simulink model "SAPF_pq0_theory"  (R2025a)
settings: Solver=VariableStepAuto  StartTime=0.0  StopTime=0.5  RelTol=1e-3
libraries: fl_lib x16, nesl_utility x16, ee_lib x12, mcbeeMathTransformLib x2, eeGeneralControl x1
settings Model: Creator=nahiz  LastModifiedBy=18023021
settings SimscapeCC: SimscapeNominalValues="[{\"value\":\"1\",\"unit\":\"A\"},{\"value\":\"1\",\"unit\":\"bar\"},{\"value\":\"1\",\"unit\":\"cm^2\"},{\"value\":\"1\",\"unit\":\"cm^3/s\"},{\"value\":\"1\",\"unit\":\"kJ/kg\"},{\"value\":\"1\",\"unit\":\"kW\"},{\"value\":\"1\",\"unit\":\"l\"},{\"value\":\"1\",\"unit\":\"N\"},{\"value\":\"1\",\"unit\":\"N*m\"},{\"value\":\"1\",\"unit\":\"V\"},{\"value\":\"0.001\",\"unit\":\"Wb\"}]"  SimscapeLogType=all  SimscapeLogDataHistory=10000.0

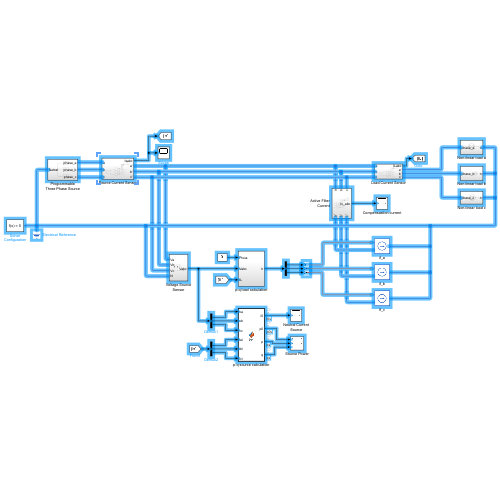
[thumbnail: Simulink's stored preview of the top-level diagram]
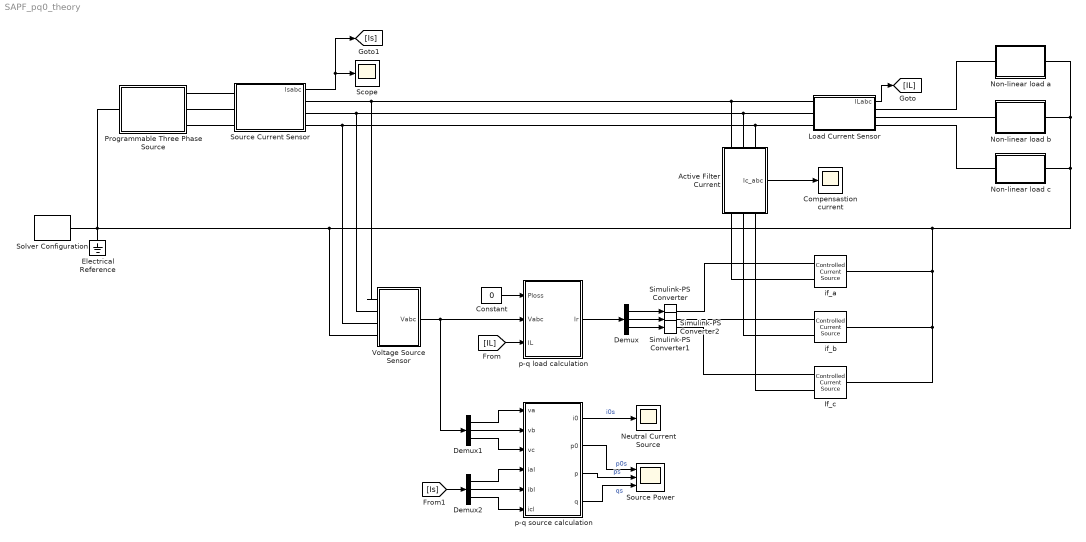
== system SAPF_pq0_theory ==
  Active Filter Current : Subsystem
      settings: PortSchema="{\"entries\":[{\"content\":{\"sides\":[{\"content\":{\"connectorIds\":[\"LConn1\",\"LConn2\",\"LConn3\"]},\"type\":\"ConnectorPlacement.EquallySpacedRectSide\",\"uuid\":\"e0b89ca1-2dce-4101-8bbe-782629a672ac\"},{\"content\":{\"connectorIds\":[\"RConn1\",\"RConn2\",\"RConn3\"],\"side\":\"RIGHT\"},\"type\":\"ConnectorPlacement.EquallySpacedRectSide\",\"uuid\":\"01d628be-6f4d-45a1-9eca-35615a86d2be\"},{\"content\":{\"side\":\"TOP\"},\"type\":\"ConnectorPlacement.EquallySpacedRectSide\",\"uuid\":\"f08109ad-0e21-41b9-b238-385b9ba1e634\"},{\"content\":{\"connectorIds\":[\"Out1\"],\"side\":\"BOTTOM\"},\"type\":\"ConnectorPlacement.EquallySpacedRectSide\",\"uuid\":\"6980f4f4-e67c-41c5-899b-6138d1e73cf4\"}]},\"type\":\"ConnectorPlacement.EquallySpacedConnector\",\"uuid\":\"23e52943-ee20-486d-b1d7-7933c9cd5a10\"}],\"packageUris\":[\"http://schema.mathworks.com/mf0/Connector/R2020b\"],\"version\":\"1.0\"}"
  Compensastion current : Scope
      settings: DataLoggingVariableName=ScopeData3
  Constant : Constant  Value=0
  Demux : Demux  Outputs=3
  Demux1 : Demux  Outputs=3
  Demux2 : Demux  Outputs=3
  Electrical Reference : fl_lib/Electrical/Electrical Elements/Electrical Reference
  If_c : fl_lib/Electrical/Electrical Sources/Controlled Current Source
  Load Current Sensor : Subsystem
  Neutral Current Source : Scope
      settings: DataLoggingVariableName=ScopeData4
  Non-linear load a : Subsystem
  Non-linear load b : Subsystem
  Non-linear load c : Subsystem
  Programmable Three Phase Source : Subsystem
  Scope : Scope
  Simulink-PS Converter : nesl_utility/Simulink-PS Converter  PhysicalDomain=network_engine_domain  SubClassName=ps_input  LeftPortType=input  RightPortType=output  PseudoPeriodic=off  Frequencies=[]  NoiseDistribution=none  NoiseParameters=[]  Unit=1  AffineConversion=off  FilteringAndDerivatives=zero  SimscapeFilterOrder=1  InputFilterTimeConstant=0.001  UdotUserProvided=0
  Simulink-PS Converter1 : nesl_utility/Simulink-PS Converter  PhysicalDomain=network_engine_domain  SubClassName=ps_input  LeftPortType=input  RightPortType=output  PseudoPeriodic=off  Frequencies=[]  NoiseDistribution=none  NoiseParameters=[]  Unit=1  AffineConversion=off  FilteringAndDerivatives=zero  SimscapeFilterOrder=1  InputFilterTimeConstant=0.001  UdotUserProvided=0
  Simulink-PS Converter2 : nesl_utility/Simulink-PS Converter  PhysicalDomain=network_engine_domain  SubClassName=ps_input  LeftPortType=input  RightPortType=output  PseudoPeriodic=off  Frequencies=[]  NoiseDistribution=none  NoiseParameters=[]  Unit=1  AffineConversion=off  FilteringAndDerivatives=zero  SimscapeFilterOrder=1  InputFilterTimeConstant=0.001  UdotUserProvided=0
  Solver Configuration : nesl_utility/Solver Configuration  PhysicalDomain=network_engine_domain  SubClassName=solver  LeftPortType=input  RightPortType=generic  Tones=[]  Harmonics=[]  SimulateNoise=off  Profile=off  UseLocalSampling=off  EnableSwitchedLinearOptims=on  FrequencyDomain=off  UseCCode=off  RelTol=0.001  AbsTol=0.001  MinStep=1e-09  ToWorkspace=off  RevertToSquareIcSolve=off  NumHomotopyIterations=100  PhasorMode=off  PhasorModeNumHarmonics=1  ConsistencySolver=NEWTON_XTOL_AFTER_FTOL  IndexReductionMethod=DerivativeReplacement  DoDC=off  ResidualTolerance=1e-09  ConsistencyTolSource=GLOBAL  ConsistencyAbsTol=0.001  ConsistencyRelTol=0.001  ConsistencyTolFactor=0.001  UseLocalSolver=off  LocalSolverChoice=NE_BACKWARD_EULER_ADVANCER  ResolveIndetEquations=on  FunctionEvalNumThread=1  LocalSolverSampleTime=0.001  DoFixedCost=off  MaxNonlinIter=3  MaxModeIter=2  ComputeImpulses=off  ImpulseIterations=2  LinearAlgebra=auto  LinearAlgebraNumThread=0  EquationFormulation=NE_TIME_EF  DelaysMemoryBudget=1024  AutomaticFiltering=on  FilteringTimeConstant=0.001  PartitionStorageMethod=AS_NEEDED  PartitionMemoryBudget=1024  PartitionMethod=ROBUST  MultibodyUseLocalSolver=off  MultibodyLocalSolverChoice=ODE1  MultibodyLocalSolverSampleTime=0.001
  Source Current Sensor : Subsystem
  Source Power : Scope  NumInputPorts=3
      settings: ActiveDisplayYMinimum=-299.915797041433  ActiveDisplayYMaximum=2699.2421733727761  DataLoggingVariableName=ScopeData2
  Voltage Source Sensor : Subsystem
  if_a : fl_lib/Electrical/Electrical Sources/Controlled Current Source
  if_b : fl_lib/Electrical/Electrical Sources/Controlled Current Source
  p-q load calculation : Subsystem
  p-q source calculation : MATLAB Function  TreatAsAtomicUnit=on
  wires:
  Load Current Sensor/1(ILabc) -> [IL]
  Source Current Sensor/1(Isabc) -> [Is], Scope/1
  Voltage Source Sensor/1(Vabc) -> Demux1/1, p-q load calculation/2(Vabc)
  p-q load calculation/1(Ir) -> Demux/1
  Constant/1 -> p-q load calculation/1(Ploss)
  [IL] -> p-q load calculation/3(IL)
  Demux/1 -> Simulink-PS Converter/1
  Demux/2 -> Simulink-PS Converter1/1
  Demux/3 -> Simulink-PS Converter2/1
  Demux1/1 -> p-q source calculation/1(va)
  Demux1/2 -> p-q source calculation/2(vb)
  Demux1/3 -> p-q source calculation/3(vc)
  [Is] -> Demux2/1
  Demux2/1 -> p-q source calculation/4(ial)
  Demux2/2 -> p-q source calculation/5(ibl)
  Demux2/3 -> p-q source calculation/6(icl)
  p-q source calculation/1(i0) -> Neutral Current Source/1  "i0s"
  p-q source calculation/2(p0) -> Source Power/1  "p0s"
  p-q source calculation/3(p) -> Source Power/2  "ps"
  p-q source calculation/4(q) -> Source Power/3  "qs"
  Active Filter Current/1(Ic_abc) -> Compensastion current/1
  connections:
  Active Filter Current/LConn3 -- Voltage Source Sensor/LConn3 -- Source Current Sensor/RConn3 -- Load Current Sensor/LConn3
  Active Filter Current/LConn2 -- Voltage Source Sensor/LConn2 -- Source Current Sensor/RConn2 -- Load Current Sensor/LConn2
  Programmable Three Phase Source/RConn1 -- Solver Configuration/RConn1 -- Electrical Reference/LConn1 -- Voltage Source Sensor/LConn4 -- Non-linear load b/RConn1 -- Non-linear load a/RConn1 -- Non-linear load c/RConn1 -- If_c/LConn1 -- if_b/LConn1 -- if_a/LConn1
  Active Filter Current/LConn1 -- Voltage Source Sensor/LConn1 -- Source Current Sensor/RConn1 -- Load Current Sensor/LConn1
  if_b/RConn2 -- Active Filter Current/RConn2
  if_a/RConn2 -- Active Filter Current/RConn1
  Programmable Three Phase Source/LConn2 -- Source Current Sensor/LConn2
  Programmable Three Phase Source/LConn1 -- Source Current Sensor/LConn1
  Programmable Three Phase Source/LConn3 -- Source Current Sensor/LConn3
  If_c/RConn2 -- Active Filter Current/RConn3
  Simulink-PS Converter/RConn1 -- if_a/RConn1
  Simulink-PS Converter1/RConn1 -- if_b/RConn1
  Simulink-PS Converter2/RConn1 -- If_c/RConn1
  Load Current Sensor/RConn3 -- Non-linear load c/LConn1
  Load Current Sensor/RConn2 -- Non-linear load b/LConn1
  Load Current Sensor/RConn1 -- Non-linear load a/LConn1

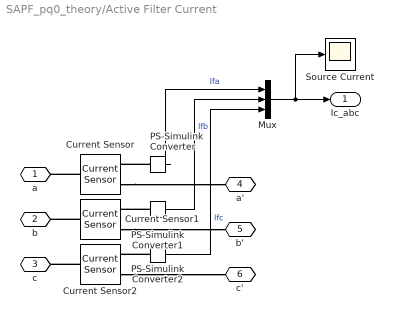
== system SAPF_pq0_theory/Active Filter Current ==
  Current Sensor : fl_lib/Electrical/Electrical Sensors/Current Sensor
  Current Sensor1 : fl_lib/Electrical/Electrical Sensors/Current Sensor
  Current Sensor2 : fl_lib/Electrical/Electrical Sensors/Current Sensor
  Mux : Mux  Inputs=3
  PS-Simulink Converter : nesl_utility/PS-Simulink Converter  PhysicalDomain=network_engine_domain  SubClassName=ps_output  LeftPortType=input  RightPortType=output  PseudoPeriodic=off  Frequencies=[]  VectorFormat=inherit  Unit=inherit  AffineConversion=off
  PS-Simulink Converter1 : nesl_utility/PS-Simulink Converter  PhysicalDomain=network_engine_domain  SubClassName=ps_output  LeftPortType=input  RightPortType=output  PseudoPeriodic=off  Frequencies=[]  VectorFormat=inherit  Unit=inherit  AffineConversion=off
  PS-Simulink Converter2 : nesl_utility/PS-Simulink Converter  PhysicalDomain=network_engine_domain  SubClassName=ps_output  LeftPortType=input  RightPortType=output  PseudoPeriodic=off  Frequencies=[]  VectorFormat=inherit  Unit=inherit  AffineConversion=off
  Source Current : Scope
  a : PMIOPort  Side=Left
  b : PMIOPort  Port=2  Side=Left
  c : PMIOPort  Port=3  Side=Left
  a' : PMIOPort  Port=4  Side=Right
  b' : PMIOPort  Port=5  Side=Right
  c' : PMIOPort  Port=6  Side=Right
  Ic_abc : Outport
  wires:
  PS-Simulink Converter1/1 -> Mux/2  "Ifb"
  PS-Simulink Converter/1 -> Mux/1  "Ifa"
  PS-Simulink Converter2/1 -> Mux/3  "Ifc"
  Mux/1 -> Source Current/1, Ic_abc/1
  connections:
  PS-Simulink Converter2/LConn1 -- Current Sensor2/RConn1
  PS-Simulink Converter1/LConn1 -- Current Sensor1/RConn1
  Current Sensor/LConn1 -- a/RConn1
  PS-Simulink Converter/LConn1 -- Current Sensor/RConn1
  Current Sensor2/LConn1 -- c/RConn1
  Current Sensor1/LConn1 -- b/RConn1
  Current Sensor/RConn2 -- a'/RConn1
  Current Sensor1/RConn2 -- b'/RConn1
  Current Sensor2/RConn2 -- c'/RConn1

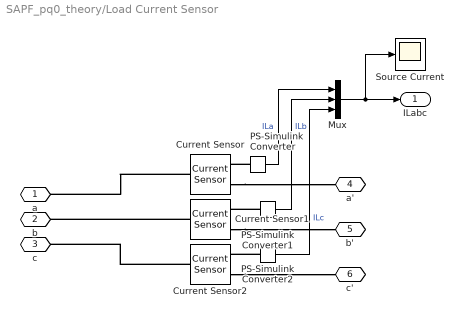
== system SAPF_pq0_theory/Load Current Sensor ==
  Current Sensor : fl_lib/Electrical/Electrical Sensors/Current Sensor
  Current Sensor1 : fl_lib/Electrical/Electrical Sensors/Current Sensor
  Current Sensor2 : fl_lib/Electrical/Electrical Sensors/Current Sensor
  Mux : Mux  Inputs=3
  PS-Simulink Converter : nesl_utility/PS-Simulink Converter  PhysicalDomain=network_engine_domain  SubClassName=ps_output  LeftPortType=input  RightPortType=output  PseudoPeriodic=off  Frequencies=[]  VectorFormat=inherit  Unit=inherit  AffineConversion=off
  PS-Simulink Converter1 : nesl_utility/PS-Simulink Converter  PhysicalDomain=network_engine_domain  SubClassName=ps_output  LeftPortType=input  RightPortType=output  PseudoPeriodic=off  Frequencies=[]  VectorFormat=inherit  Unit=inherit  AffineConversion=off
  PS-Simulink Converter2 : nesl_utility/PS-Simulink Converter  PhysicalDomain=network_engine_domain  SubClassName=ps_output  LeftPortType=input  RightPortType=output  PseudoPeriodic=off  Frequencies=[]  VectorFormat=inherit  Unit=inherit  AffineConversion=off
  Source Current : Scope
  a : PMIOPort  Side=Left
  b : PMIOPort  Port=2  Side=Left
  c : PMIOPort  Port=3  Side=Left
  a' : PMIOPort  Port=4  Side=Right
  b' : PMIOPort  Port=5  Side=Right
  c' : PMIOPort  Port=6  Side=Right
  ILabc : Outport
  wires:
  PS-Simulink Converter1/1 -> Mux/2  "ILb"
  PS-Simulink Converter/1 -> Mux/1  "ILa"
  PS-Simulink Converter2/1 -> Mux/3  "ILc"
  Mux/1 -> Source Current/1, ILabc/1
  connections:
  PS-Simulink Converter2/LConn1 -- Current Sensor2/RConn1
  PS-Simulink Converter1/LConn1 -- Current Sensor1/RConn1
  Current Sensor/LConn1 -- a/RConn1
  PS-Simulink Converter/LConn1 -- Current Sensor/RConn1
  Current Sensor2/LConn1 -- c/RConn1
  Current Sensor1/LConn1 -- b/RConn1
  Current Sensor/RConn2 -- a'/RConn1
  Current Sensor1/RConn2 -- b'/RConn1
  Current Sensor2/RConn2 -- c'/RConn1

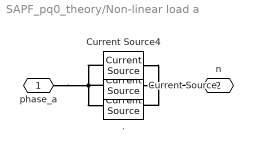
== system SAPF_pq0_theory/Non-linear load a ==
  . : ee_lib/Sources/Current Source  dc_current=0 A  ac_current=1 A  ac_shift=10 deg  ac_frequency=7*50 Hz  noise_mode=ee.enum.sources.noise.Disabled  PSD=0 A^2/Hz  sample_time=1e-3 s  repeatability=ee.enum.sources.repeatability.NotRepeatable  user_seed=0  auto_seed=3516351732  i_specify=off  i_priority=None  i=0 A  i_nominal_specify=off  i_nominal_value=1  i_nominal_unit=A  v_specify=off  v_priority=None  v=0 V  v_nominal_specify=off  v_nominal_value=1  v_nominal_unit=V
  Current Source : ee_lib/Sources/Current Source  dc_current=0 A  ac_current=20 A  ac_shift=10 deg  ac_frequency=50 Hz  noise_mode=ee.enum.sources.noise.Disabled  PSD=0 A^2/Hz  sample_time=1e-3 s  repeatability=ee.enum.sources.repeatability.NotRepeatable  user_seed=0  auto_seed=3127860819  i_specify=off  i_priority=None  i=0 A  i_nominal_specify=off  i_nominal_value=1  i_nominal_unit=A  v_specify=off  v_priority=None  v=0 V  v_nominal_specify=off  v_nominal_value=1  v_nominal_unit=V
  Current Source4 : ee_lib/Sources/Current Source  dc_current=0 A  ac_current=3 A  ac_shift=10 deg  ac_frequency=5*50 Hz  noise_mode=ee.enum.sources.noise.Disabled  PSD=0 A^2/Hz  sample_time=1e-3 s  repeatability=ee.enum.sources.repeatability.NotRepeatable  user_seed=0  auto_seed=810846759  i_specify=off  i_priority=None  i=0 A  i_nominal_specify=off  i_nominal_value=1  i_nominal_unit=A  v_specify=off  v_priority=None  v=0 V  v_nominal_specify=off  v_nominal_value=1  v_nominal_unit=V
  phase_a : PMIOPort  Side=Left
  n : PMIOPort  Port=2  Side=Right
  connections:
  Current Source/LConn1 -- ./LConn1 -- n/RConn1 -- Current Source4/LConn1
  Current Source4/RConn1 -- ./RConn1 -- phase_a/RConn1 -- Current Source/RConn1

== system SAPF_pq0_theory/Non-linear load b ==
  Current Source5 : ee_lib/Sources/Current Source  dc_current=0 A  ac_current=20 A  ac_shift=-130 deg  ac_frequency=50 Hz  noise_mode=ee.enum.sources.noise.Disabled  PSD=0 A^2/Hz  sample_time=1e-3 s  repeatability=ee.enum.sources.repeatability.NotRepeatable  user_seed=0  auto_seed=5147076  i_specify=off  i_priority=None  i=0 A  i_nominal_specify=off  i_nominal_value=1  i_nominal_unit=A  v_specify=off  v_priority=None  v=0 V  v_nominal_specify=off  v_nominal_value=1  v_nominal_unit=V
  Current Source6 : ee_lib/Sources/Current Source  dc_current=0 A  ac_current=1 A  ac_shift=-130 deg  ac_frequency=7*50 Hz  noise_mode=ee.enum.sources.noise.Disabled  PSD=0 A^2/Hz  sample_time=1e-3 s  repeatability=ee.enum.sources.repeatability.NotRepeatable  user_seed=0  auto_seed=1359011463  i_specify=off  i_priority=None  i=0 A  i_nominal_specify=off  i_nominal_value=1  i_nominal_unit=A  v_specify=off  v_priority=None  v=0 V  v_nominal_specify=off  v_nominal_value=1  v_nominal_unit=V
  Current Source7 : ee_lib/Sources/Current Source  dc_current=0 A  ac_current=3 A  ac_shift=-130 deg  ac_frequency=5*50 Hz  noise_mode=ee.enum.sources.noise.Disabled  PSD=0 A^2/Hz  sample_time=1e-3 s  repeatability=ee.enum.sources.repeatability.NotRepeatable  user_seed=0  auto_seed=3004832076  i_specify=off  i_priority=None  i=0 A  i_nominal_specify=off  i_nominal_value=1  i_nominal_unit=A  v_specify=off  v_priority=None  v=0 V  v_nominal_specify=off  v_nominal_value=1  v_nominal_unit=V
  phase_b : PMIOPort  Side=Left
  n : PMIOPort  Port=2  Side=Right
  connections:
  Current Source6/LConn1 -- n/RConn1 -- Current Source7/LConn1 -- Current Source5/LConn1
  Current Source6/RConn1 -- phase_b/RConn1 -- Current Source7/RConn1 -- Current Source5/RConn1

== system SAPF_pq0_theory/Non-linear load c ==
  Current Source1 : ee_lib/Sources/Current Source  dc_current=0 A  ac_current=3 A  ac_shift=110 deg  ac_frequency=5*50 Hz  noise_mode=ee.enum.sources.noise.Disabled  PSD=0 A^2/Hz  sample_time=1e-3 s  repeatability=ee.enum.sources.repeatability.NotRepeatable  user_seed=0  auto_seed=755105624  i_specify=off  i_priority=None  i=0 A  i_nominal_specify=off  i_nominal_value=1  i_nominal_unit=A  v_specify=off  v_priority=None  v=0 V  v_nominal_specify=off  v_nominal_value=1  v_nominal_unit=V
  Current Source2 : ee_lib/Sources/Current Source  dc_current=0 A  ac_current=20 A  ac_shift=110 deg  ac_frequency=50 Hz  noise_mode=ee.enum.sources.noise.Disabled  PSD=0 A^2/Hz  sample_time=1e-3 s  repeatability=ee.enum.sources.repeatability.NotRepeatable  user_seed=0  auto_seed=1547781561  i_specify=off  i_priority=None  i=0 A  i_nominal_specify=off  i_nominal_value=1  i_nominal_unit=A  v_specify=off  v_priority=None  v=0 V  v_nominal_specify=off  v_nominal_value=1  v_nominal_unit=V
  Current Source8 : ee_lib/Sources/Current Source  dc_current=0 A  ac_current=1 A  ac_shift=110 deg  ac_frequency=7*50 Hz  noise_mode=ee.enum.sources.noise.Disabled  PSD=0 A^2/Hz  sample_time=1e-3 s  repeatability=ee.enum.sources.repeatability.NotRepeatable  user_seed=0  auto_seed=2685450550  i_specify=off  i_priority=None  i=0 A  i_nominal_specify=off  i_nominal_value=1  i_nominal_unit=A  v_specify=off  v_priority=None  v=0 V  v_nominal_specify=off  v_nominal_value=1  v_nominal_unit=V
  phase_c : PMIOPort  Side=Left
  n : PMIOPort  Port=2  Side=Right
  connections:
  Current Source8/LConn1 -- Current Source1/LConn1 -- n/RConn1 -- Current Source2/LConn1
  Current Source1/RConn1 -- phase_c/RConn1 -- Current Source8/RConn1 -- Current Source2/RConn1

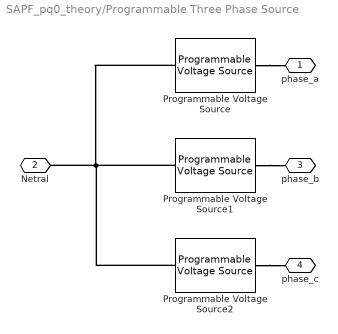
== system SAPF_pq0_theory/Programmable Three Phase Source ==
  Programmable Voltage Source : ee_lib/Sources/Programmable Voltage Source  magnitude_type=ee.enum.timechanging.constant  ac_magnitude=100 V  magn_ramp=1 V/s  magn_step=1 V  magn_modu_magn=1 V  magn_modu_freq=1 Hz  magn_t1=1 s  magn_t2=2 s  frequency_type=ee.enum.timechanging.constant  ac_frequency=50 Hz  freq_ramp=1 Hz/s  freq_step=1 Hz  freq_modu_magn=1 Hz  freq_modu_freq=1 Hz  freq_t1=1 s  freq_t2=2 s  phase_type=ee.enum.timechanging.constant  ac_shift=0 deg  phase_ramp=1 deg/s  phase_step=1 deg  phase_modu_magn=1 deg  phase_modu_freq=1 Hz  phase_t1=1 s  phase_t2=2 s  dc_type=ee.enum.timechanging.constant  dc_voltage=0 V  dc_ramp=1 V/s  dc_step=1 V  dc_modu_magn=1 V  dc_modu_freq=1 Hz  dc_t1=1 s  dc_t2=2 s  harmonic_option=1  harmonic_orders=[5, 7, 11, 13]  harmonic_ratios=[.2, .2, .1, .1]  harmonic_shifts=[0, 0, 0, 0] deg  harmonic_t1=-inf s  harmonic_t2=inf s  noise_mode=0  PSD=0 V^2/Hz  repeatability=1  auto_seed=0  user_seed=0  sample_time=1e-3 s  i_specify=off  i_priority=None  i=0 A  i_nominal_specify=off  i_nominal_value=1  i_nominal_unit=A  v_specify=off  v_priority=None  v=0 V  v_nominal_specify=off  v_nominal_value=1  v_nominal_unit=V
      settings: InternalSimscapePortConfiguration="{\"Bottom\":[],\"Left\":[{\"id\":\"p\",\"label\":\"+\",\"type\":\"foundation.electrical.electrical\"}],\"Right\":[{\"id\":\"n\",\"label\":\"-\",\"type\":\"foundation.electrical.electrical\"}],\"Top\":[]}"
  Programmable Voltage Source1 : ee_lib/Sources/Programmable Voltage Source  magnitude_type=ee.enum.timechanging.constant  ac_magnitude=311 V  magn_ramp=1 V/s  magn_step=1 V  magn_modu_magn=1 V  magn_modu_freq=1 Hz  magn_t1=1 s  magn_t2=2 s  frequency_type=ee.enum.timechanging.constant  ac_frequency=50 Hz  freq_ramp=1 Hz/s  freq_step=1 Hz  freq_modu_magn=1 Hz  freq_modu_freq=1 Hz  freq_t1=1 s  freq_t2=2 s  phase_type=ee.enum.timechanging.constant  ac_shift=-120 deg  phase_ramp=1 deg/s  phase_step=1 deg  phase_modu_magn=1 deg  phase_modu_freq=1 Hz  phase_t1=1 s  phase_t2=2 s  dc_type=ee.enum.timechanging.constant  dc_voltage=0 V  dc_ramp=1 V/s  dc_step=1 V  dc_modu_magn=1 V  dc_modu_freq=1 Hz  dc_t1=1 s  dc_t2=2 s  harmonic_option=1  harmonic_orders=[5, 7, 11, 13]  harmonic_ratios=[.2, .2, .1, .1]  harmonic_shifts=[0, 0, 0, 0] deg  harmonic_t1=-inf s  harmonic_t2=inf s  noise_mode=0  PSD=0 V^2/Hz  repeatability=1  auto_seed=0  user_seed=0  sample_time=1e-3 s  i_specify=off  i_priority=None  i=0 A  i_nominal_specify=off  i_nominal_value=1  i_nominal_unit=A  v_specify=off  v_priority=None  v=0 V  v_nominal_specify=off  v_nominal_value=1  v_nominal_unit=V
      settings: InternalSimscapePortConfiguration="{\"Bottom\":[],\"Left\":[{\"id\":\"p\",\"label\":\"+\",\"type\":\"foundation.electrical.electrical\"}],\"Right\":[{\"id\":\"n\",\"label\":\"-\",\"type\":\"foundation.electrical.electrical\"}],\"Top\":[]}"
  Programmable Voltage Source2 : ee_lib/Sources/Programmable Voltage Source  magnitude_type=ee.enum.timechanging.constant  ac_magnitude=311 V  magn_ramp=1 V/s  magn_step=1 V  magn_modu_magn=1 V  magn_modu_freq=1 Hz  magn_t1=1 s  magn_t2=2 s  frequency_type=ee.enum.timechanging.constant  ac_frequency=50 Hz  freq_ramp=1 Hz/s  freq_step=1 Hz  freq_modu_magn=1 Hz  freq_modu_freq=1 Hz  freq_t1=1 s  freq_t2=2 s  phase_type=ee.enum.timechanging.constant  ac_shift=120 deg  phase_ramp=1 deg/s  phase_step=1 deg  phase_modu_magn=1 deg  phase_modu_freq=1 Hz  phase_t1=1 s  phase_t2=2 s  dc_type=ee.enum.timechanging.constant  dc_voltage=0 V  dc_ramp=1 V/s  dc_step=1 V  dc_modu_magn=1 V  dc_modu_freq=1 Hz  dc_t1=1 s  dc_t2=2 s  harmonic_option=1  harmonic_orders=[5, 7, 11, 13]  harmonic_ratios=[.2, .2, .1, .1]  harmonic_shifts=[0, 0, 0, 0] deg  harmonic_t1=-inf s  harmonic_t2=inf s  noise_mode=0  PSD=0 V^2/Hz  repeatability=1  auto_seed=0  user_seed=0  sample_time=1e-3 s  i_specify=off  i_priority=None  i=0 A  i_nominal_specify=off  i_nominal_value=1  i_nominal_unit=A  v_specify=off  v_priority=None  v=0 V  v_nominal_specify=off  v_nominal_value=1  v_nominal_unit=V
      settings: InternalSimscapePortConfiguration="{\"Bottom\":[],\"Left\":[{\"id\":\"p\",\"label\":\"+\",\"type\":\"foundation.electrical.electrical\"}],\"Right\":[{\"id\":\"n\",\"label\":\"-\",\"type\":\"foundation.electrical.electrical\"}],\"Top\":[]}"
  phase_a : PMIOPort  Side=Left
  Netral : PMIOPort  Port=2  Side=Right
  phase_b : PMIOPort  Port=3  Side=Left
  phase_c : PMIOPort  Port=4  Side=Left
  connections:
  Programmable Voltage Source2/LConn1 -- phase_c/RConn1
  Programmable Voltage Source1/RConn1 -- Programmable Voltage Source2/RConn1 -- Programmable Voltage Source/RConn1 -- Netral/RConn1
  Programmable Voltage Source/LConn1 -- phase_a/RConn1
  Programmable Voltage Source1/LConn1 -- phase_b/RConn1

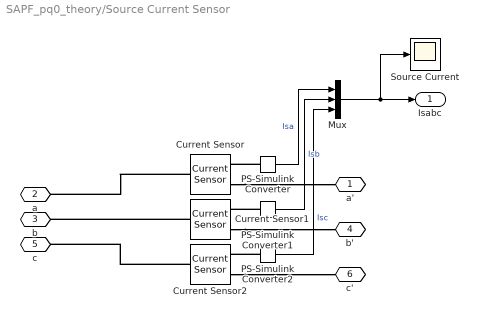
== system SAPF_pq0_theory/Source Current Sensor ==
  Current Sensor : fl_lib/Electrical/Electrical Sensors/Current Sensor
  Current Sensor1 : fl_lib/Electrical/Electrical Sensors/Current Sensor
  Current Sensor2 : fl_lib/Electrical/Electrical Sensors/Current Sensor
  Mux : Mux  Inputs=3
  PS-Simulink Converter : nesl_utility/PS-Simulink Converter  PhysicalDomain=network_engine_domain  SubClassName=ps_output  LeftPortType=input  RightPortType=output  PseudoPeriodic=off  Frequencies=[]  VectorFormat=inherit  Unit=inherit  AffineConversion=off
  PS-Simulink Converter1 : nesl_utility/PS-Simulink Converter  PhysicalDomain=network_engine_domain  SubClassName=ps_output  LeftPortType=input  RightPortType=output  PseudoPeriodic=off  Frequencies=[]  VectorFormat=inherit  Unit=inherit  AffineConversion=off
  PS-Simulink Converter2 : nesl_utility/PS-Simulink Converter  PhysicalDomain=network_engine_domain  SubClassName=ps_output  LeftPortType=input  RightPortType=output  PseudoPeriodic=off  Frequencies=[]  VectorFormat=inherit  Unit=inherit  AffineConversion=off
  Source Current : Scope
  a' : PMIOPort  Side=Right
  a : PMIOPort  Port=2  Side=Left
  b : PMIOPort  Port=3  Side=Left
  b' : PMIOPort  Port=4  Side=Right
  c : PMIOPort  Port=5  Side=Left
  c' : PMIOPort  Port=6  Side=Right
  Isabc : Outport
  wires:
  PS-Simulink Converter1/1 -> Mux/2  "Isb"
  PS-Simulink Converter/1 -> Mux/1  "Isa"
  PS-Simulink Converter2/1 -> Mux/3  "Isc"
  Mux/1 -> Source Current/1, Isabc/1
  connections:
  PS-Simulink Converter2/LConn1 -- Current Sensor2/RConn1
  PS-Simulink Converter1/LConn1 -- Current Sensor1/RConn1
  Current Sensor/LConn1 -- a/RConn1
  PS-Simulink Converter/LConn1 -- Current Sensor/RConn1
  Current Sensor2/LConn1 -- c/RConn1
  Current Sensor1/LConn1 -- b/RConn1
  Current Sensor/RConn2 -- a'/RConn1
  Current Sensor1/RConn2 -- b'/RConn1
  Current Sensor2/RConn2 -- c'/RConn1

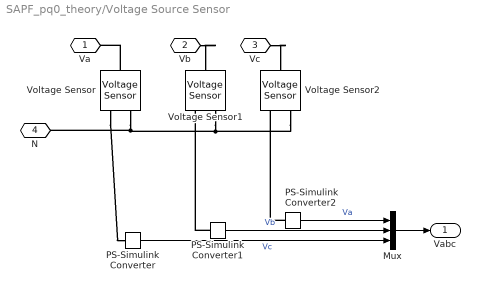
== system SAPF_pq0_theory/Voltage Source Sensor ==
  Mux : Mux  Inputs=3
  PS-Simulink Converter : nesl_utility/PS-Simulink Converter  PhysicalDomain=network_engine_domain  SubClassName=ps_output  LeftPortType=input  RightPortType=output  PseudoPeriodic=off  Frequencies=[]  VectorFormat=inherit  Unit=inherit  AffineConversion=off
  PS-Simulink Converter1 : nesl_utility/PS-Simulink Converter  PhysicalDomain=network_engine_domain  SubClassName=ps_output  LeftPortType=input  RightPortType=output  PseudoPeriodic=off  Frequencies=[]  VectorFormat=inherit  Unit=inherit  AffineConversion=off
  PS-Simulink Converter2 : nesl_utility/PS-Simulink Converter  PhysicalDomain=network_engine_domain  SubClassName=ps_output  LeftPortType=input  RightPortType=output  PseudoPeriodic=off  Frequencies=[]  VectorFormat=inherit  Unit=inherit  AffineConversion=off
  Voltage Sensor : fl_lib/Electrical/Electrical Sensors/Voltage Sensor
  Voltage Sensor1 : fl_lib/Electrical/Electrical Sensors/Voltage Sensor
  Voltage Sensor2 : fl_lib/Electrical/Electrical Sensors/Voltage Sensor
  Va : PMIOPort  Side=Left
  Vb : PMIOPort  Port=2  Side=Left
  Vc : PMIOPort  Port=3  Side=Left
  N : PMIOPort  Port=4  Side=Left
  Vabc : Outport
  wires:
  PS-Simulink Converter/1 -> Mux/3  "Vc"
  PS-Simulink Converter2/1 -> Mux/1  "Va"
  PS-Simulink Converter1/1 -> Mux/2  "Vb"
  Mux/1 -> Vabc/1
  connections:
  PS-Simulink Converter1/LConn1 -- Voltage Sensor1/RConn1
  Voltage Sensor1/RConn2 -- Voltage Sensor2/RConn2 -- Voltage Sensor/RConn2 -- N/RConn1
  Voltage Sensor/RConn1 -- PS-Simulink Converter/LConn1
  PS-Simulink Converter2/LConn1 -- Voltage Sensor2/RConn1
  Voltage Sensor/LConn1 -- Va/RConn1
  Vb/RConn1 -- Voltage Sensor1/LConn1
  Vc/RConn1 -- Voltage Sensor2/LConn1

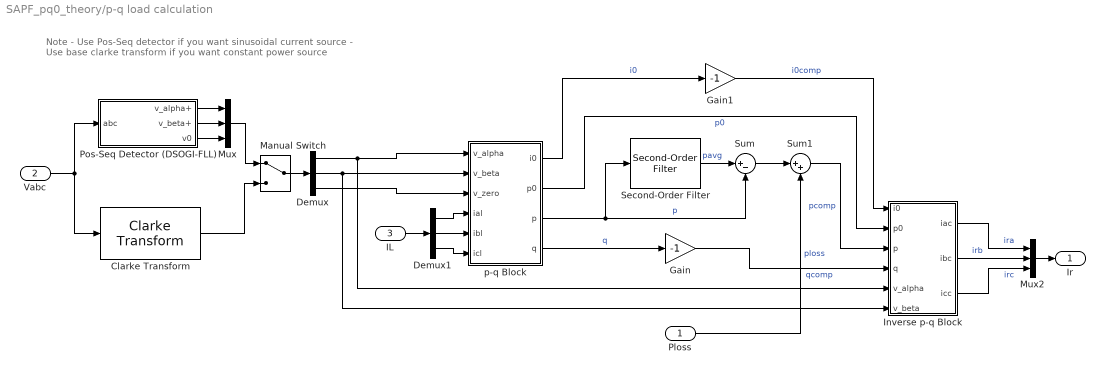
== system SAPF_pq0_theory/p-q load calculation ==
  note: Note
      | - Use Pos-Seq detector if you want sinusoidal current source
      | - Use base clarke transform if you want constant power source
  Ploss : Inport
  Vabc : Inport  Port=2
  IL : Inport  Port=3
  Clarke Transform : mcbeeMathTransformLib/Clarke Transform  PowerInvariant=on  UseWithEmbedded=off  PhaseInput=Two inputs
      settings: LibrarySourceBlock=|
      | ee_sl_lib/Mathematical
      | Transforms/Clarke Transform
  Demux : Demux  Outputs=3
  Demux1 : Demux  Outputs=3
  Gain : Gain  Gain=-1
  Gain1 : Gain  Gain=-1
  Inverse p-q Block : MATLAB Function  TreatAsAtomicUnit=on
  Manual Switch : ManualSwitch
  Mux : Mux  Inputs=3
  Mux2 : Mux  Inputs=3
  Pos-Seq Detector (DSOGI-FLL) : Subsystem
  Second-Order Filter : eeGeneralControl/Second-Order Filter  FilterType=Low-pass  fn=5  Zeta=1  Ts=-1  A0=0  Ph0=0  f0=0  b0=0
      settings: LibrarySourceBlock=ee_sl_lib/General Control/Second-Order Filter
  Sum : Sum  Inputs=|+-
  Sum1 : Sum  Inputs=|++
  p-q Block : MATLAB Function  TreatAsAtomicUnit=on
  Ir : Outport
  wires:
  Inverse p-q Block/3(icc) -> Mux2/3  "irc"
  IL/1 -> Demux1/1
  Demux1/2 -> p-q Block/5(ibl)
  Mux2/1 -> Ir/1
  Inverse p-q Block/1(iac) -> Mux2/1  "ira"
  Demux1/1 -> p-q Block/4(ial)
  Inverse p-q Block/2(ibc) -> Mux2/2  "irb"
  p-q Block/1(i0) -> Gain1/1  "i0"
  p-q Block/3(p) -> Second-Order Filter/1, Sum/2  "p"
  Ploss/1 -> Sum1/2  "ploss"
  Second-Order Filter/1 -> Sum/1  "pavg"
  Sum/1 -> Sum1/1
  Sum1/1 -> Inverse p-q Block/3(p)  "pcomp"
  p-q Block/4(q) -> Gain/1  "q"
  Demux1/3 -> p-q Block/6(icl)
  p-q Block/2(p0) -> Inverse p-q Block/2(p0)  "p0"
  Gain/1 -> Inverse p-q Block/4(q)  "qcomp"
  Gain1/1 -> Inverse p-q Block/1(i0)  "i0comp"
  Vabc/1 -> Clarke Transform/1, Pos-Seq Detector (DSOGI-FLL)/1(abc)
  Demux/1 -> Inverse p-q Block/5(v_alpha), p-q Block/1(v_alpha)
  Demux/3 -> p-q Block/3(v_zero)
  Clarke Transform/1 -> Manual Switch/2
  Pos-Seq Detector (DSOGI-FLL)/1(v_alpha+) -> Mux/1
  Pos-Seq Detector (DSOGI-FLL)/2(v_beta+) -> Mux/2
  Pos-Seq Detector (DSOGI-FLL)/3(v0) -> Mux/3
  Demux/2 -> Inverse p-q Block/6(v_beta), p-q Block/2(v_beta)
  Mux/1 -> Manual Switch/1
  Manual Switch/1 -> Demux/1

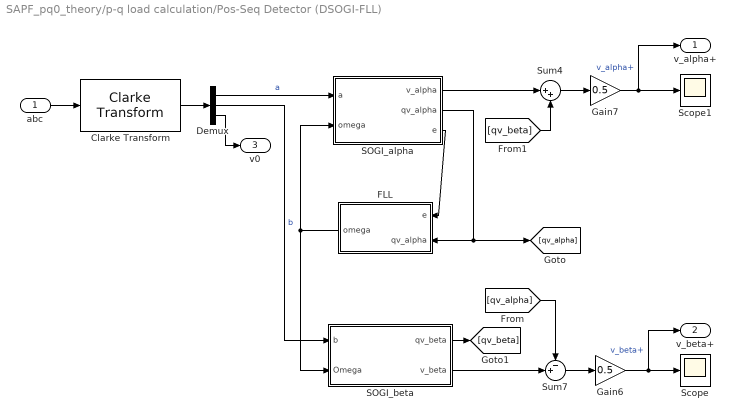
== system SAPF_pq0_theory/p-q load calculation/Pos-Seq Detector (DSOGI-FLL) ==
  abc : Inport
  Clarke Transform : mcbeeMathTransformLib/Clarke Transform  PowerInvariant=on  UseWithEmbedded=off  PhaseInput=Two inputs
      settings: LibrarySourceBlock=|
      | ee_sl_lib/Mathematical
      | Transforms/Clarke Transform
  Demux : Demux  Outputs=3
  FLL : Subsystem
  Gain6 : Gain  Gain=0.5
  Gain7 : Gain  Gain=0.5
  SOGI_alpha : Subsystem
  SOGI_beta : Subsystem
  Scope : Scope
      settings: ActiveDisplayYMinimum=-1  ActiveDisplayYMaximum=1  DataLoggingVariableName=ScopeData6
  Scope1 : Scope
      settings: DataLoggingVariableName=ScopeData5
  Sum4 : Sum  Inputs=|++
  Sum7 : Sum  Inputs=-+|
  v_alpha+ : Outport
  v_beta+ : Outport  Port=2
  v0 : Outport  Port=3
  wires:
  Sum4/1 -> Gain7/1
  Sum7/1 -> Gain6/1
  abc/1 -> Clarke Transform/1
  Gain6/1 -> Scope/1, v_beta+/1  "v_beta+"
  Demux/3 -> v0/1
  [qv_alpha] -> Sum7/1
  Clarke Transform/1 -> Demux/1
  Gain7/1 -> Scope1/1, v_alpha+/1  "v_alpha+"
  [qv_beta] -> Sum4/2
  SOGI_alpha/2(qv_alpha) -> [qv_alpha], FLL/2(qv_alpha)
  Demux/1 -> SOGI_alpha/1(a)  "a"
  SOGI_alpha/1(v_alpha) -> Sum4/1
  FLL/1(omega) -> SOGI_beta/2(Omega), SOGI_alpha/2(omega)
  SOGI_alpha/3(e) -> FLL/1(e)
  Demux/2 -> SOGI_beta/1(b)  "b"
  SOGI_beta/1(qv_beta) -> [qv_beta]
  SOGI_beta/2(v_beta) -> Sum7/2

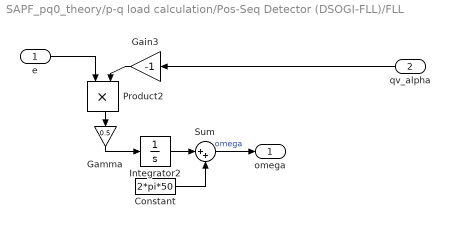
== system SAPF_pq0_theory/p-q load calculation/Pos-Seq Detector (DSOGI-FLL)/FLL ==
  e : Inport
  qv_alpha : Inport  Port=2
  Constant : Constant  Value=2*pi*50
  Gain3 : Gain  Gain=-1
  Gamma : Gain  Gain=0.5
  Integrator2 : Integrator
  Product2 : Product
  Sum : Sum  Inputs=|++
  omega : Outport
  wires:
  Sum/1 -> omega/1  "omega"
  Gamma/1 -> Integrator2/1
  Gain3/1 -> Product2/2
  Product2/1 -> Gamma/1
  Constant/1 -> Sum/2
  qv_alpha/1 -> Gain3/1
  Integrator2/1 -> Sum/1
  e/1 -> Product2/1

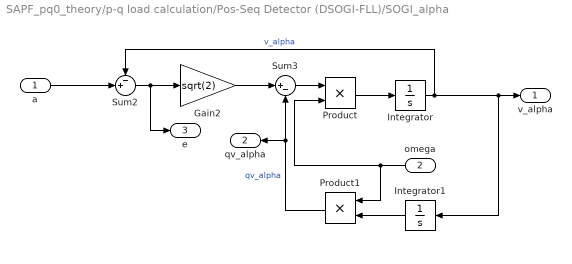
== system SAPF_pq0_theory/p-q load calculation/Pos-Seq Detector (DSOGI-FLL)/SOGI_alpha ==
  a : Inport
  omega : Inport  Port=2
  Gain2 : Gain  Gain=sqrt(2)
  Integrator : Integrator
  Integrator1 : Integrator
  Product : Product
  Product1 : Product
  Sum2 : Sum  Inputs=-+|
  Sum3 : Sum  Inputs=|+-
  v_alpha : Outport
  qv_alpha : Outport  Port=2
  e : Outport  Port=3
  wires:
  a/1 -> Sum2/2
  Sum2/1 -> e/1, Gain2/1
  Product/1 -> Integrator/1
  Gain2/1 -> Sum3/1
  Integrator1/1 -> Product1/2
  Sum3/1 -> Product/1
  Integrator/1 -> v_alpha/1, Integrator1/1, Sum2/1  "v_alpha"
  Product1/1 -> Sum3/2, qv_alpha/1  "qv_alpha"
  omega/1 -> Product1/1, Product/2

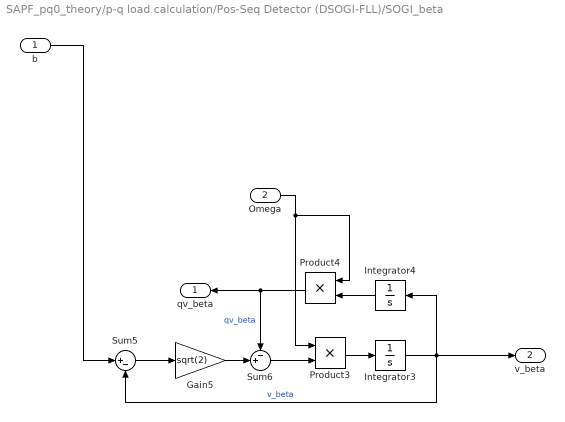
== system SAPF_pq0_theory/p-q load calculation/Pos-Seq Detector (DSOGI-FLL)/SOGI_beta ==
  b : Inport
  Omega : Inport  Port=2
  Gain5 : Gain  Gain=sqrt(2)
  Integrator3 : Integrator
  Integrator4 : Integrator
  Product3 : Product
  Product4 : Product
  Sum5 : Sum  Inputs=|+-
  Sum6 : Sum  Inputs=-+|
  qv_beta : Outport
  v_beta : Outport  Port=2
  wires:
  Integrator4/1 -> Product4/2
  Product4/1 -> qv_beta/1, Sum6/1  "qv_beta"
  Omega/1 -> Product4/1, Product3/1
  Integrator3/1 -> v_beta/1, Sum5/2, Integrator4/1  "v_beta"
  Gain5/1 -> Sum6/2
  Sum5/1 -> Gain5/1
  Product3/1 -> Integrator3/1
  Sum6/1 -> Product3/2
  b/1 -> Sum5/1

== matlab function SAPF_pq0_theory/p-q load calculation/Inverse p-q Block ==
  data: i0 input; p0 input; p input; iac output; q input; v_alpha input; v_beta input; ibc output; icc output

function [iac,ibc,icc] = fcn(i0,p0,p,q,v_alpha, v_beta)
%#codegen
%% Zero Sequence Current
i_zero = i0;
%% Voltage Threshold Protection
Vph_rms_nom = 220;
Vab_min = 0.05*sqrt(3/2)*sqrt(2)*Vph_rms_nom;
D_min = Vab_min^2;
%% Denominator
D = v_alpha^2 + v_beta^2;
%% Inverse p-q Calculation
if D > D_min
    i_alpha = (v_alpha*p + v_beta*q)/D;
    i_beta = (v_beta*p - v_alpha*q)/D;
else
    % Prevent division by near-zero voltage
    i_alpha = 0;
    i_beta  = 0;
end
%% Inverse Clarke Transformation
iac = sqrt(2/3)*(i_zero/sqrt(2)+i_alpha);
ibc = sqrt(2/3)*(i_zero/sqrt(2)-i_alpha/2 ...
     + sqrt(3)*i_beta/2);
icc = sqrt(2/3)*(i_zero/sqrt(2)-i_alpha/2 ...
     - sqrt(3)*i_beta/2);
end

== matlab function SAPF_pq0_theory/p-q load calculation/p-q Block ==
  data: i0 output; p0 output; v_alpha input; p output; v_beta input; v_zero input; ial input; ibl input; icl input; q output
function [i0,p0,p,q]= fcn(v_alpha,v_beta, v_zero,ial,ibl,icl)
%#codegen
il_zero=(ial+ibl+icl)/sqrt(3);
il_alpha=(ial-ibl/2-icl/2)*sqrt(2/3);
il_beta=(ibl-icl)/sqrt(2);
i0=il_zero;
p0=v_zero.*il_zero;
p=v_alpha.*il_alpha+v_beta.*il_beta;
q=v_beta.*il_alpha-v_alpha.*il_beta;

== matlab function SAPF_pq0_theory/p-q source calculation ==
  data: i0 output; p0 output; va input; p output; vb input; vc input; ial input; ibl input; icl input; q output
function [i0,p0,p,q]= fcn(va,vb,vc,ial,ibl,icl)
%#codegen
v_zero=(va+vb+vc)/sqrt(3);
v_alpha=(va-vb/2-vc/2)*sqrt(2/3);
v_beta=(vb-vc)/sqrt(2);
il_zero=(ial+ibl+icl)/sqrt(3);
il_alpha=(ial-ibl/2-icl/2)*sqrt(2/3);
il_beta=(ibl-icl)/sqrt(2);
i0=il_zero;
p0=v_zero.*il_zero;
p=v_alpha.*il_alpha+v_beta.*il_beta;
q=v_beta.*il_alpha-v_alpha.*il_beta;
